simulink model "Swing_UP_esther"  (R2025a)
settings: Solver=ode4  StartTime=0.0  StopTime=100  FixedStep=0.0005  RelTol=1e-3
InitFcn:
  | addpath('functions');
model workspace (MATLAB code in the model file):
  | arm_torque = 0;
  | L_arm = 0.2;
  | I_arm = 0.01;
  | lcom_1 = 0.6;
  | I_1 = 0.02;
  | m_1 = 1;
  | L_1 = 1;
  | g = 9.81;
  | 
  | init_cond = [0; 0; pi; 0];
  | fric_arm = [0, 0, 0];
  | fric_1 = [0, 0, 0];
undefined symbols (not defined in the file or in its folder): quantization_interval, sampling_time, v_theta_1_LPF_gain, v_theta_arm_LPF_gain
settings Model: Creator=Esther  LastModifiedBy=Esther

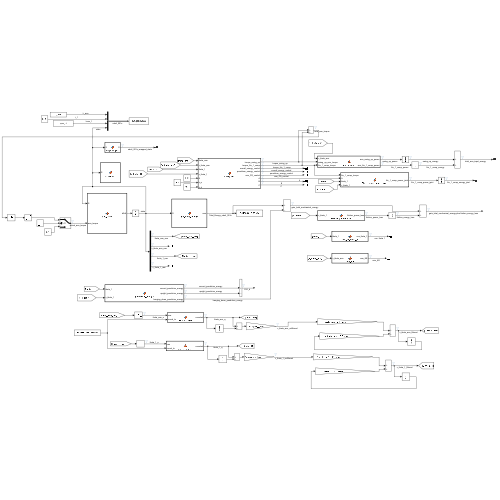
[thumbnail: Simulink's stored preview of the top-level diagram]
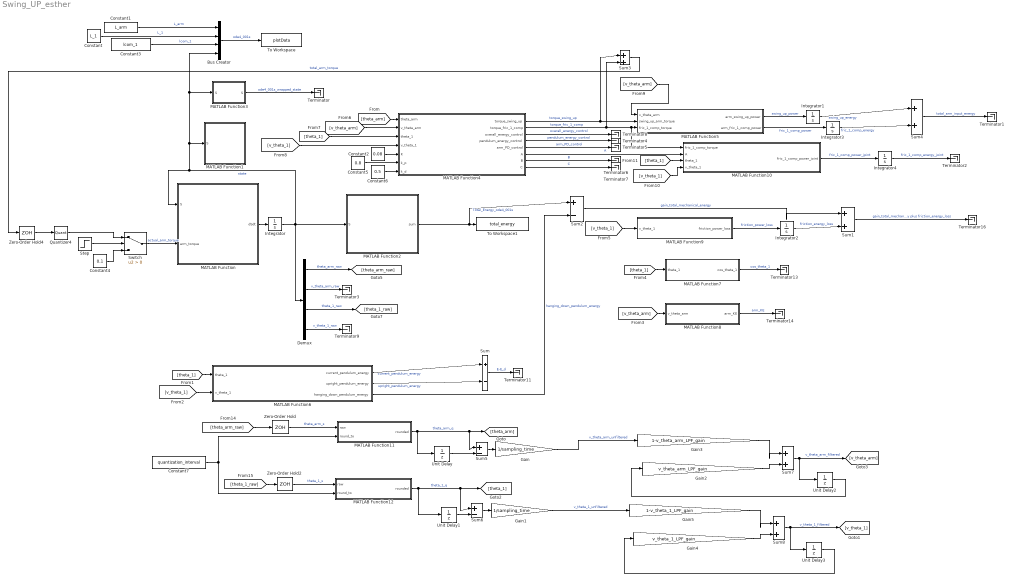
== system Swing_UP_esther ==
  Bus Creator : BusCreator  Inputs=4
  Constant : Constant  Value=L_1
  Constant1 : Constant  Value=L_arm
  Constant2 : Constant  Value=0.08
  Constant3 : Constant  Value=lcom_1
  Constant4 : Constant  Value=0.1
  Constant5 : Constant  Value=0.8
  Constant6 : Constant  Value=0.5
  Constant7 : Constant  Value=quantization_interval
  Demux : Demux
  Gain : Gain  Gain=1/sampling_time
  Gain1 : Gain  Gain=1/sampling_time
  Gain2 : Gain  Gain=v_theta_arm_LPF_gain
  Gain3 : Gain  Gain=1-v_theta_arm_LPF_gain
  Gain4 : Gain  Gain=v_theta_1_LPF_gain
  Gain5 : Gain  Gain=1-v_theta_1_LPF_gain
  Integrator : Integrator  InitialCondition=init_cond
  Integrator{1..4} (4 alike) : Integrator
  MATLAB Function : MATLAB Function  TreatAsAtomicUnit=on
  MATLAB Function1 : MATLAB Function  TreatAsAtomicUnit=on
  MATLAB Function10 : MATLAB Function  TreatAsAtomicUnit=on
  MATLAB Function11 : MATLAB Function  TreatAsAtomicUnit=on
  MATLAB Function12 : MATLAB Function  TreatAsAtomicUnit=on
  MATLAB Function2 : MATLAB Function  TreatAsAtomicUnit=on
  MATLAB Function3 : MATLAB Function  TreatAsAtomicUnit=on
  MATLAB Function4 : MATLAB Function  TreatAsAtomicUnit=on
  MATLAB Function5 : MATLAB Function  TreatAsAtomicUnit=on
  MATLAB Function6 : MATLAB Function  TreatAsAtomicUnit=on
  MATLAB Function7 : MATLAB Function  TreatAsAtomicUnit=on
  MATLAB Function8 : MATLAB Function  TreatAsAtomicUnit=on
  MATLAB Function9 : MATLAB Function  TreatAsAtomicUnit=on
  Quantizer4 : Quantizer  QuantizationInterval=quantization_interval
  Step : Step  Time=0.05  SampleTime=0
  Sum{,2,5..6} (4 alike) : Sum  Inputs=|+-
  Sum{1,3..4,7..8} (5 alike) : Sum  Inputs=|++
  Switch : Switch  Criteria=u2 > Threshold  SaturateOnIntegerOverflow=off  InputSameDT=off
  Terminator{,1..9,11,13..14,16} (14 alike) : Terminator
  To Workspace : ToWorkspace  VariableName=plotData  SaveFormat=Timeseries  SampleTime=-1
  To Workspace1 : ToWorkspace  VariableName=total_energy  SaveFormat=Timeseries  SampleTime=-1
  Unit Delay : UnitDelay  SampleTime=sampling_time  HasFrameUpgradeWarning=on
  Unit Delay1 : UnitDelay  InitialCondition=pi  SampleTime=sampling_time  HasFrameUpgradeWarning=on
  Unit Delay2 : UnitDelay  SampleTime=sampling_time  HasFrameUpgradeWarning=on
  Unit Delay3 : UnitDelay  SampleTime=sampling_time  HasFrameUpgradeWarning=on
  Zero-Order Hold : ZeroOrderHold  SampleTime=sampling_time
  Zero-Order Hold2 : ZeroOrderHold  SampleTime=sampling_time
  Zero-Order Hold4 : ZeroOrderHold  SampleTime=sampling_time
  wires:
  MATLAB Function/1(dSdt) -> Integrator/1
  Constant1/1 -> Bus Creator/1  "L_arm"
  Constant3/1 -> Bus Creator/3  "lcom_1"
  Integrator/1 -> MATLAB Function2/1(S), MATLAB Function1/1(S), Bus Creator/4, MATLAB Function3/1("S "), MATLAB Function/1(S), Demux/1  "state"
  Bus Creator/1 -> To Workspace/1  "ode4_001s"
  Constant/1 -> Bus Creator/2  "L_1"
  MATLAB Function2/1(sum) -> Sum2/1, To Workspace1/1  "Total_Energy_ode4_001s"
  MATLAB Function3/1(S) -> Terminator/1  "ode4_001s_wrapped_state"
  Constant2/1 -> MATLAB Function4/5(K)
  MATLAB Function4/1(torque_swing_up) -> Sum3/1, MATLAB Function5/2(swing_up_arm_torque)  "torque_swing_up"
  Constant5/1 -> MATLAB Function4/6(k_p)
  Constant6/1 -> MATLAB Function4/7(k_d)
  MATLAB Function4/6(A) -> MATLAB Function10/2(A)  "A"
  MATLAB Function5/1(arm_swing_up_power) -> Integrator1/1  "swing_up_power"
  Integrator1/1 -> Sum4/1  "swing_up_energy"
  MATLAB Function4/4(pendulum_energy_control) -> Terminator4/1  "pendulum_energy_control"
  MATLAB Function4/5(arm_PD_control) -> Terminator5/1  "arm_PD_control"
  MATLAB Function4/7(B) -> Terminator6/1  "B"
  MATLAB Function4/8(C) -> Terminator7/1  "C"
  MATLAB Function4/3(overall_energy_control) -> Terminator8/1  "overall_energy_control"
  MATLAB Function6/1(current_pendulum_energy) -> Sum/1  "current_pendulum_energy"
  MATLAB Function6/2(upright_pendulum_energy) -> Sum/2  "upright_pendulum_energy"
  Sum/1 -> Terminator11/1  "E-E_d"
  MATLAB Function7/1(cos_theta_1) -> Terminator13/1  "cos_theta_1"
  MATLAB Function8/1(arm_KE) -> Terminator14/1  "arm_KE"
  MATLAB Function9/1(friction_power_loss) -> Integrator2/1  "friction_power_loss"
  Integrator2/1 -> Sum1/2  "friction_energy_loss"
  Sum1/1 -> Terminator16/1  "gain_total_mechanical_energy plus friction_energy_loss"
  MATLAB Function6/3(hanging_down_pendulum_energy) -> Sum2/2  "hanging_down_pendulum_energy"
  MATLAB Function4/2(torque_fric_1_comp) -> MATLAB Function10/1(fric_1_comp_torque), MATLAB Function5/3(fric_1_comp_torque), Sum3/2  "torque_fric_1_comp"
  Sum3/1 -> Zero-Order Hold4/1  "total_arm_torque"
  MATLAB Function5/2(arm_fric_1_comp_power) -> Integrator3/1  "fric_1_comp_power"
  Integrator3/1 -> Sum4/2  "fric_1_comp_energy"
  Sum4/1 -> Terminator1/1  "total_arm_input_energy"
  Demux/1 -> [theta_arm_raw]  "theta_arm_raw"
  Demux/3 -> [theta_1_raw]  "theta_1_raw"
  Demux/4 -> Terminator9/1  "v_theta_1_raw"
  Sum2/1 -> Sum1/1  "gain_total_mechanical_energy"
  [theta_1] -> MATLAB Function6/1(theta_1)
  [v_theta_1] -> MATLAB Function6/2(v_theta_1)
  [v_theta_arm] -> MATLAB Function8/1(v_theta_arm)
  [theta_1] -> MATLAB Function7/1(theta_1)
  [v_theta_1] -> MATLAB Function9/1(v_theta_1)
  [theta_arm] -> MATLAB Function4/1(theta_arm)
  [v_theta_arm] -> MATLAB Function4/2(v_theta_arm)
  [theta_1] -> MATLAB Function4/3(theta_1)
  [v_theta_1] -> MATLAB Function4/4(v_theta_1)
  [v_theta_arm] -> MATLAB Function5/1(v_theta_arm)
  MATLAB Function10/1(fric_1_comp_power_joint) -> Integrator4/1  "fric_1_comp_power_jpint"
  Integrator4/1 -> Terminator2/1  "fric_1_comp_energy_joint"
  [v_theta_1] -> MATLAB Function10/4(v_theta_1)
  [theta_1] -> MATLAB Function10/3(theta_1)
  Demux/2 -> Terminator3/1  "v_theta_arm_raw"
  Zero-Order Hold4/1 -> Quantizer4/1
  Quantizer4/1 -> Switch/1
  Switch/1 -> MATLAB Function/2(arm_torque)  "actual_arm_torque"
  Constant4/1 -> Switch/3
  Step/1 -> Switch/2
  Gain3/1 -> Sum7/1
  Gain2/1 -> Sum7/2
  Sum7/1 -> Unit Delay2/1, [v_theta_arm]  "v_theta_arm_filtered"
  Unit Delay2/1 -> Gain2/1
  Gain4/1 -> Sum8/2
  Sum8/1 -> Unit Delay3/1, [v_theta_1]  "v_theta_1_filtered"
  Unit Delay3/1 -> Gain4/1
  Gain5/1 -> Sum8/1
  Constant7/1 -> MATLAB Function11/2(round_to), MATLAB Function12/2(round_to)
  MATLAB Function11/1(rounded) -> Sum5/1, [theta_arm], Unit Delay/1  "theta_arm_q"
  Zero-Order Hold/1 -> MATLAB Function11/1(raw)  "theta_arm_s"
  [theta_arm_raw] -> Zero-Order Hold/1
  Unit Delay/1 -> Sum5/2
  Sum5/1 -> Gain/1
  Gain/1 -> Gain3/1  "v_theta_arm_unfiltered"
  Zero-Order Hold2/1 -> MATLAB Function12/1(raw)  "theta_1_s"
  Sum6/1 -> Gain1/1
  Gain1/1 -> Gain5/1  "v_theta_1_unfiltered"
  Unit Delay1/1 -> Sum6/2
  MATLAB Function12/1(rounded) -> Unit Delay1/1, Sum6/1, [theta_1]  "theta_1_q"
  [theta_1_raw] -> Zero-Order Hold2/1

== matlab function Swing_UP_esther/MATLAB Function5 ==
  data: v_theta_arm input; arm_swing_up_power output; swing_up_arm_torque input; fric_1_comp_torque input; arm_fric_1_comp_power output
function [arm_swing_up_power, arm_fric_1_comp_power] = arm_power(v_theta_arm, swing_up_arm_torque, fric_1_comp_torque)
    arm_swing_up_power = v_theta_arm*swing_up_arm_torque;
    arm_fric_1_comp_power = v_theta_arm*fric_1_comp_torque;
end

== matlab function Swing_UP_esther/MATLAB Function6 ==
  data: theta_1 input; v_theta_1 input; m_1 parameter size=1; current_pendulum_energy output size=1; lcom_1 parameter size=1; I_1 parameter size=1; g parameter size=1; upright_pendulum_energy output; hanging_down_pendulum_energy output
function [current_pendulum_energy, upright_pendulum_energy, hanging_down_pendulum_energy] = pendulum_energy(theta_1, v_theta_1, m_1, lcom_1, I_1, g)
    current_pendulum_energy = (1/2)*(m_1*lcom_1^2+I_1)*v_theta_1^2 + m_1*g*lcom_1*cos(theta_1); % only the pendulum is considered (ignoring effect from the arm)
    upright_pendulum_energy = m_1*g*lcom_1;
    hanging_down_pendulum_energy = -m_1*g*lcom_1;
end

== matlab function Swing_UP_esther/MATLAB Function7 ==
  data: theta_1 input; cos_theta_1 output
function cos_theta_1 = cos_of_theta_1(theta_1)
    cos_theta_1 = cos(theta_1);
end

== matlab function Swing_UP_esther/MATLAB Function8 ==
  data: arm_KE output; v_theta_arm input; I_arm parameter size=1
function arm_KE = arm_KE(v_theta_arm, I_arm)
    arm_KE = (1/2)*I_arm*v_theta_arm^2;
end

== matlab function Swing_UP_esther/MATLAB Function9 ==
  data: friction_power_loss output; v_theta_1 input; fric_1 parameter size=[1 3]
function friction_power_loss = friction_power_loss(v_theta_1, fric_1)
    friction_power_loss = fric_1(1, 1)*v_theta_1^2 + fric_1(1, 2)*tanh(fric_1(1, 3)*abs(v_theta_1))*abs(v_theta_1);
end

== matlab function Swing_UP_esther/MATLAB Function10 ==
  data: fric_1_comp_torque input; A input; fric_1_comp_power_joint output; theta_1 input; v_theta_1 input; m_1 parameter size=1; L_arm parameter size=1; lcom_1 parameter size=1
function fric_1_comp_power_joint = fric_1_comp_power_joint(fric_1_comp_torque, A, theta_1, v_theta_1, m_1, L_arm, lcom_1)

    torque_fric_1_comp_joint = -fric_1_comp_torque*m_1*L_arm*lcom_1*cos(theta_1)/A;
    fric_1_comp_power_joint = torque_fric_1_comp_joint*v_theta_1;
end

== matlab function Swing_UP_esther/MATLAB Function11 ==
  data: raw input; rounded output; round_to input
function rounded = round_angle(raw, round_to)
    rounded = raw/round_to;
    rounded = round(rounded);
    rounded = rounded*round_to;
end

== matlab function Swing_UP_esther/MATLAB Function12 ==
  data: raw input; rounded output; round_to input
function rounded = round_angle(raw, round_to)
    rounded = raw/round_to;
    rounded = round(rounded);
    rounded = rounded*round_to;
end

== matlab function Swing_UP_esther/MATLAB Function1 ==
  settings: updateMethod=DISCRETE
  data: S input; L_arm parameter; L_1 parameter; lcom_1 parameter
function animation(S, L_arm, L_1, lcom_1)
    update_ratio = 100;
    realtime_animation_single(S, L_arm, L_1, lcom_1, update_ratio);
end

== matlab function Swing_UP_esther/MATLAB Function ==
  data: S input size=4; dSdt output size=4; arm_torque input size=1; L_arm parameter size=1; I_arm parameter size=1; lcom_1 parameter size=1; I_1 parameter size=1; m_1 parameter size=1; fric_arm parameter size=[1 3]; fric_1 parameter size=[1 3]; g parameter size=1
function dSdt = get_dSdt(S, arm_torque, L_arm, I_arm, lcom_1, I_1, m_1, fric_arm, fric_1, g)
    t = 0;
    phys_param = [L_arm, I_arm, lcom_1, I_1, m_1, g];
    dSdt = furuta_single_state_derivative(t, S, arm_torque, phys_param, fric_arm, fric_1);
end

== matlab function Swing_UP_esther/MATLAB Function2 ==
  data: S input size=4; sum output size=1; L_arm parameter size=1; I_arm parameter size=1; lcom_1 parameter size=1; I_1 parameter size=1; m_1 parameter size=1; g parameter size=1
function sum = get_total_energy(S, L_arm, I_arm, lcom_1, I_1, m_1, g)
    t = 0;
    phys_param = [L_arm, I_arm, lcom_1, I_1, m_1, g];
    [T_total, P_total] = furuta_single_KE_PE(t, S, phys_param);
    sum = T_total + P_total;
end

== matlab function Swing_UP_esther/MATLAB Function3 ==
  data: S input size=4; S output size=4
function S = wrap_angles(S)
    S(1) = wrapTo180(rad2deg(S(1)));
    S(3) = wrapTo180(rad2deg(S(3)));
end

== matlab function Swing_UP_esther/MATLAB Function4 ==
  settings: updateMethod=DISCRETE
  data: L_arm parameter size=1; I_arm parameter size=1; lcom_1 parameter size=1; I_1 parameter size=1; m_1 parameter size=1; g parameter size=1; theta_arm input; v_theta_arm input; theta_1 input; v_theta_1 input; torque_swing_up output; torque_fric_1_comp output; overall_energy_control output; pendulum_energy_control output; arm_PD_control output; K input; k_p input; k_d input; A output; fric_arm parameter size=[1 3]; fric_1 parameter size=[1 3]; B output; C output
function [torque_swing_up, torque_fric_1_comp, overall_energy_control, pendulum_energy_control, arm_PD_control, A, B, C] = swing_up(L_arm, I_arm, lcom_1, I_1, m_1, g, theta_arm, v_theta_arm, theta_1, v_theta_1, K, k_p, k_d, fric_arm, fric_1)
    % arm_acc_required = single_swing_up_energy_controller(L_arm, I_arm, lcom_1, I_1, m_1, g, K, theta_1, v_theta_1);
    [overall_energy_control, pendulum_energy_control, arm_PD_control] = single_swing_up_energy_controller(L_arm, I_arm, lcom_1, I_1, m_1, g, theta_arm, v_theta_arm, theta_1, v_theta_1, K, k_p, k_d);
    % arm_acc_required = arm_acc_required - k_p*theta_arm - k_d*v_theta_arm;
    [torque_swing_up, torque_fric_1_comp, A, B, C] = single_swing_up_feedback_linearisation_controller(L_arm, I_arm, lcom_1, I_1, m_1, g, theta_1, v_theta_1, v_theta_arm, fric_arm, fric_1, overall_energy_control);
end
